simulink model "t_type_three_phase_four_wire_average"  (R2025b)
settings: Solver=ode23tb  StartTime=0.0  StopTime=t_stop_3ph  MaxStep=1e-5  RelTol=1e-3
PreLoadFcn:
  | demo_root=fileparts(fileparts(get_param(bdroot,'FileName'))); run(fullfile(demo_root,'parameters','three_phase_demo_parameters.m')); clear demo_root;
undefined symbols (not defined in the file): A_lcl_3ph, B_lcl_3ph, C_lcl_3ph, D_lcl_3ph, I_ref_pk_3ph, Kdist_3ph, Kp_3ph, Kr_3ph, Ksin3_3ph, phase_shift_3ph, sin3_enable_3ph, suppression_effect_enable_3ph, V_grid_pk_3ph, Vdc_sw, w_grid_sw, wc_3ph
settings Model: Creator=bob  LastModifiedBy=bob

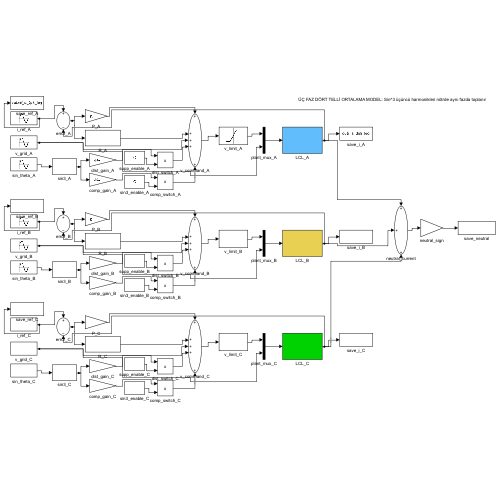
[thumbnail: Simulink's stored preview of the top-level diagram]
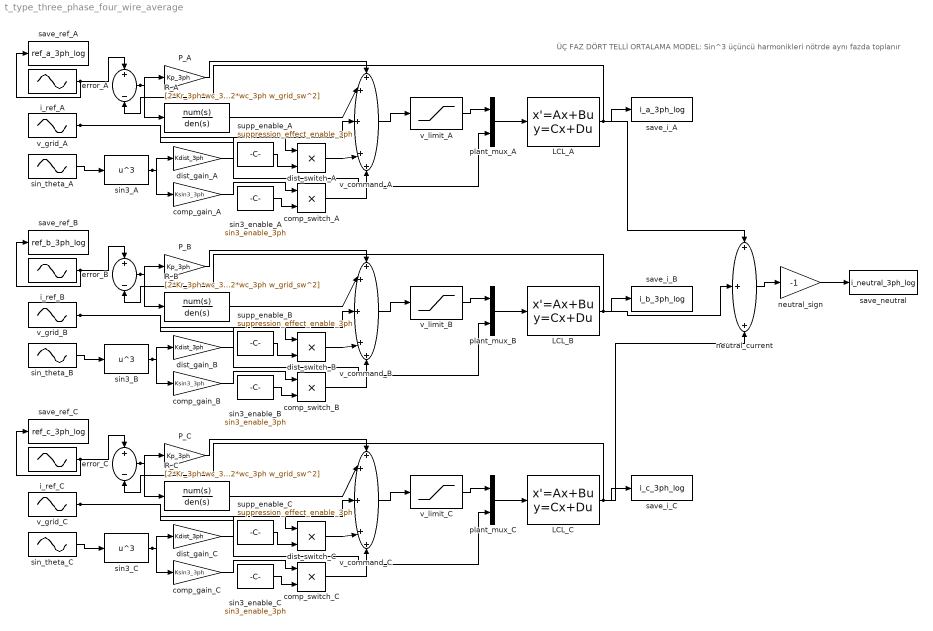
== system t_type_three_phase_four_wire_average ==
  note: ÜÇ FAZ DÖRT TELLİ ORTALAMA MODEL: Sin^3 üçüncü harmonikleri nötrde aynı fazda toplanır
  LCL_A : StateSpace  A=A_lcl_3ph  B=B_lcl_3ph  C=C_lcl_3ph  D=D_lcl_3ph  InitialCondition=[0 0 0]
  LCL_B : StateSpace  A=A_lcl_3ph  B=B_lcl_3ph  C=C_lcl_3ph  D=D_lcl_3ph  InitialCondition=[0 0 0]
  LCL_C : StateSpace  A=A_lcl_3ph  B=B_lcl_3ph  C=C_lcl_3ph  D=D_lcl_3ph  InitialCondition=[0 0 0]
  P_A : Gain  Gain=Kp_3ph
  P_B : Gain  Gain=Kp_3ph
  P_C : Gain  Gain=Kp_3ph
  R_A : TransferFcn  Numerator=[2*Kr_3ph*wc_3ph 0]  Denominator=[1 2*wc_3ph w_grid_sw^2]
  R_B : TransferFcn  Numerator=[2*Kr_3ph*wc_3ph 0]  Denominator=[1 2*wc_3ph w_grid_sw^2]
  R_C : TransferFcn  Numerator=[2*Kr_3ph*wc_3ph 0]  Denominator=[1 2*wc_3ph w_grid_sw^2]
  comp_gain_A : Gain  Gain=Ksin3_3ph
  comp_gain_B : Gain  Gain=Ksin3_3ph
  comp_gain_C : Gain  Gain=Ksin3_3ph
  comp_switch_A : Product
  comp_switch_B : Product
  comp_switch_C : Product
  dist_gain_A : Gain  Gain=Kdist_3ph
  dist_gain_B : Gain  Gain=Kdist_3ph
  dist_gain_C : Gain  Gain=Kdist_3ph
  dist_switch_A : Product
  dist_switch_B : Product
  dist_switch_C : Product
  error_A : Sum  Inputs=+-
  error_B : Sum  Inputs=+-
  error_C : Sum  Inputs=+-
  i_ref_A : Sin  Amplitude=I_ref_pk_3ph  Frequency=w_grid_sw  Phase=phase_shift_3ph(1)  SampleTime=0
  i_ref_B : Sin  Amplitude=I_ref_pk_3ph  Frequency=w_grid_sw  Phase=phase_shift_3ph(2)  SampleTime=0
  i_ref_C : Sin  Amplitude=I_ref_pk_3ph  Frequency=w_grid_sw  Phase=phase_shift_3ph(3)  SampleTime=0
  neutral_current : Sum  Inputs=+++
  neutral_sign : Gain  Gain=-1
  plant_mux_A : Mux  Inputs=2
  plant_mux_B : Mux  Inputs=2
  plant_mux_C : Mux  Inputs=2
  save_i_A : ToWorkspace  VariableName=i_a_3ph_log  SaveFormat=Timeseries  SampleTime=-1
  save_i_B : ToWorkspace  VariableName=i_b_3ph_log  SaveFormat=Timeseries  SampleTime=-1
  save_i_C : ToWorkspace  VariableName=i_c_3ph_log  SaveFormat=Timeseries  SampleTime=-1
  save_neutral : ToWorkspace  VariableName=i_neutral_3ph_log  SaveFormat=Timeseries  SampleTime=-1
  save_ref_A : ToWorkspace  VariableName=ref_a_3ph_log  SaveFormat=Timeseries  SampleTime=-1
  save_ref_B : ToWorkspace  VariableName=ref_b_3ph_log  SaveFormat=Timeseries  SampleTime=-1
  save_ref_C : ToWorkspace  VariableName=ref_c_3ph_log  SaveFormat=Timeseries  SampleTime=-1
  sin3_A : Fcn  Expr=u^3
  sin3_B : Fcn  Expr=u^3
  sin3_C : Fcn  Expr=u^3
  sin3_enable_A : Constant  Value=sin3_enable_3ph
  sin3_enable_B : Constant  Value=sin3_enable_3ph
  sin3_enable_C : Constant  Value=sin3_enable_3ph
  sin_theta_A : Sin  Frequency=w_grid_sw  Phase=phase_shift_3ph(1)  SampleTime=0
  sin_theta_B : Sin  Frequency=w_grid_sw  Phase=phase_shift_3ph(2)  SampleTime=0
  sin_theta_C : Sin  Frequency=w_grid_sw  Phase=phase_shift_3ph(3)  SampleTime=0
  supp_enable_A : Constant  Value=suppression_effect_enable_3ph
  supp_enable_B : Constant  Value=suppression_effect_enable_3ph
  supp_enable_C : Constant  Value=suppression_effect_enable_3ph
  v_command_A : Sum  Inputs=+++++
  v_command_B : Sum  Inputs=+++++
  v_command_C : Sum  Inputs=+++++
  v_grid_A : Sin  Amplitude=V_grid_pk_3ph  Frequency=w_grid_sw  Phase=phase_shift_3ph(1)  SampleTime=0
  v_grid_B : Sin  Amplitude=V_grid_pk_3ph  Frequency=w_grid_sw  Phase=phase_shift_3ph(2)  SampleTime=0
  v_grid_C : Sin  Amplitude=V_grid_pk_3ph  Frequency=w_grid_sw  Phase=phase_shift_3ph(3)  SampleTime=0
  v_limit_A : Saturate  UpperLimit=Vdc_sw/2  LowerLimit=-Vdc_sw/2
  v_limit_B : Saturate  UpperLimit=Vdc_sw/2  LowerLimit=-Vdc_sw/2
  v_limit_C : Saturate  UpperLimit=Vdc_sw/2  LowerLimit=-Vdc_sw/2
  wires:
  i_ref_A/1 -> error_A/1, save_ref_A/1
  LCL_A/1 -> error_A/2, save_i_A/1, neutral_current/1
  error_A/1 -> P_A/1, R_A/1
  sin_theta_A/1 -> sin3_A/1
  sin3_A/1 -> dist_gain_A/1, comp_gain_A/1
  dist_gain_A/1 -> dist_switch_A/1
  supp_enable_A/1 -> dist_switch_A/2
  comp_gain_A/1 -> comp_switch_A/1
  sin3_enable_A/1 -> comp_switch_A/2
  P_A/1 -> v_command_A/1
  R_A/1 -> v_command_A/2
  v_grid_A/1 -> v_command_A/3, plant_mux_A/2
  dist_switch_A/1 -> v_command_A/4
  comp_switch_A/1 -> v_command_A/5
  v_command_A/1 -> v_limit_A/1
  v_limit_A/1 -> plant_mux_A/1
  plant_mux_A/1 -> LCL_A/1
  i_ref_B/1 -> error_B/1, save_ref_B/1
  LCL_B/1 -> error_B/2, save_i_B/1, neutral_current/2
  error_B/1 -> P_B/1, R_B/1
  sin_theta_B/1 -> sin3_B/1
  sin3_B/1 -> dist_gain_B/1, comp_gain_B/1
  dist_gain_B/1 -> dist_switch_B/1
  supp_enable_B/1 -> dist_switch_B/2
  comp_gain_B/1 -> comp_switch_B/1
  sin3_enable_B/1 -> comp_switch_B/2
  P_B/1 -> v_command_B/1
  R_B/1 -> v_command_B/2
  v_grid_B/1 -> v_command_B/3, plant_mux_B/2
  dist_switch_B/1 -> v_command_B/4
  comp_switch_B/1 -> v_command_B/5
  v_command_B/1 -> v_limit_B/1
  v_limit_B/1 -> plant_mux_B/1
  plant_mux_B/1 -> LCL_B/1
  i_ref_C/1 -> error_C/1, save_ref_C/1
  LCL_C/1 -> error_C/2, save_i_C/1, neutral_current/3
  error_C/1 -> P_C/1, R_C/1
  sin_theta_C/1 -> sin3_C/1
  sin3_C/1 -> dist_gain_C/1, comp_gain_C/1
  dist_gain_C/1 -> dist_switch_C/1
  supp_enable_C/1 -> dist_switch_C/2
  comp_gain_C/1 -> comp_switch_C/1
  sin3_enable_C/1 -> comp_switch_C/2
  P_C/1 -> v_command_C/1
  R_C/1 -> v_command_C/2
  v_grid_C/1 -> v_command_C/3, plant_mux_C/2
  dist_switch_C/1 -> v_command_C/4
  comp_switch_C/1 -> v_command_C/5
  v_command_C/1 -> v_limit_C/1
  v_limit_C/1 -> plant_mux_C/1
  plant_mux_C/1 -> LCL_C/1
  neutral_current/1 -> neutral_sign/1
  neutral_sign/1 -> save_neutral/1
